simulink model "Unbalanced_Fault_Analysis"  (R2024a)
settings: Solver=VariableStepAuto  StartTime=0.0  StopTime=0.5  RelTol=1e-3
libraries: spsThreePhasePISectionLineLib x2, spsThreePhaseVIMeasurementLib x2, spsThreePhaseParallelRLCLoadLib x1, spsThreePhaseFaultLib x1, spsThreePhaseSourceLib x1, sps_lib x1
settings Model: Creator=Naman V Shetty  LastModifiedBy=Naman V Shetty

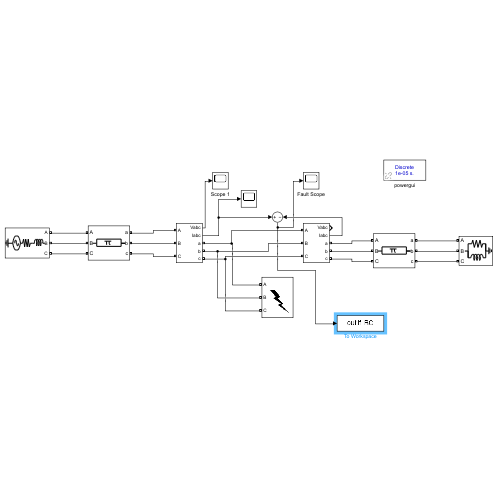
[thumbnail: Simulink's stored preview of the top-level diagram]
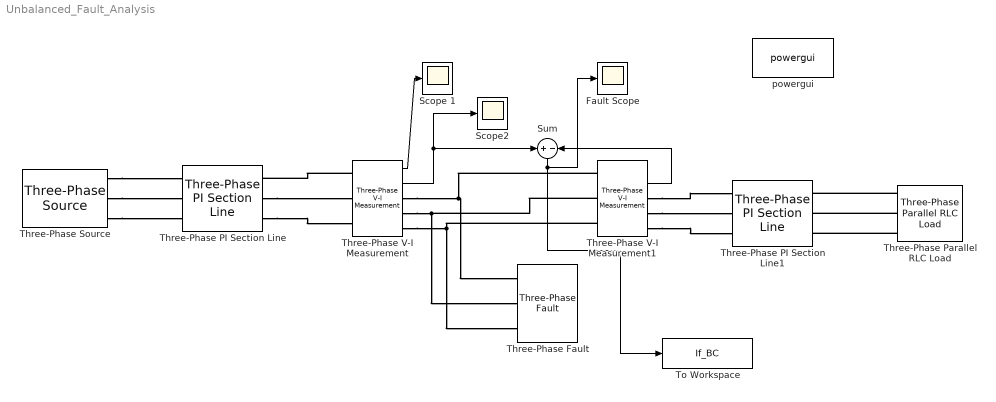
== system Unbalanced_Fault_Analysis ==
  Fault Scope : Scope
  Scope 1 : Scope
      settings: Tag=Voltage
  Scope2 : Scope
  Sum : Sum  Inputs=+-
  Three-Phase PI Section Line : spsThreePhasePISectionLineLib/Three-Phase PI Section Line  LConnTagsString=a|b|c  RConnTagsString=A|B|C  Length=25  Frequency=50  Resistances=[0.2 0.6]  Inductances=[0.001 0.003]  Capacitances=[12e-9 6e-9]
  Three-Phase PI Section Line1 : spsThreePhasePISectionLineLib/Three-Phase PI Section Line  LConnTagsString=a|b|c  RConnTagsString=A|B|C  Length=25  Frequency=50  Resistances=[0.2 0.6]  Inductances=[0.001 0.003]  Capacitances=[12e-9 6e-9]
  Three-Phase Parallel RLC Load : spsThreePhaseParallelRLCLoadLib/Three-Phase Parallel RLC Load  LConnTagsString=A|B|C  Configuration=Y (grounded)  NominalVoltage=11000  Vabc=[1e3 1e3 1e3]  Vabcp=[1e3 1e3 1e3]  NominalFrequency=50  UnbalancedPower=off  ActivePower=1.5e6  InductivePower=0.5e6  CapacitivePower=0  Pabc=[10e3 9e3 11e3]  QLabc=[100 90 110]  QCabc=[100 90 110]  Pabcp=[10e3 9e3 11e3]  QLabcp=[100 90 110]  QCabcp=[100 90 110]  Measurements=None  LoadType=constant Z
  Three-Phase V-I Measurement : spsThreePhaseVIMeasurementLib/Three-Phase V-I Measurement  VoltageMeasurement=phase-to-ground  SetLabelV=off  LabelV=Vabc  Vpu=off  VpuLL=off  CurrentMeasurement=yes  SetLabelI=off  LabelI=Iabc  Ipu=off  Pbase=100e6  Vbase=500e3  OutputType=Complex  PhasorSimulation=off  PSBequivalent=0
  Three-Phase V-I Measurement1 : spsThreePhaseVIMeasurementLib/Three-Phase V-I Measurement  VoltageMeasurement=phase-to-ground  SetLabelV=off  LabelV=Vabc  Vpu=off  VpuLL=off  CurrentMeasurement=yes  SetLabelI=off  LabelI=Iabc  Ipu=off  Pbase=100e6  Vbase=500e3  OutputType=Complex  PhasorSimulation=off  PSBequivalent=0
  Three-Phase Fault : spsThreePhaseFaultLib/Three-Phase Fault  InitialStates=0  FaultA=off  FaultB=on  FaultC=on  GroundFault=off  SwitchTimes=[0.1 0.3]  External=off  SwitchStatus=NaN  FaultResistance=0.01  GroundResistance=0.01  SnubberResistance=1e6  SnubberCapacitance=inf  Measurements=None
  Three-Phase Source : spsThreePhaseSourceLib/Three-Phase Source  InternalConnection=Yg  VoltagePhases=off  Voltage=11000  PhaseAngle=0  Voltage_phases=[25e3 25e3 25e3]/sqrt(3)  PhaseAngles_phases=[0 -120 +120]  Frequency=50  NonIdealSource=on  SpecifyImpedance=off  Resistance=0.1  Inductance=0.001  ShortCircuitLevel=100e6  BaseVoltage=11e3  XRratio=7  BusType=swing  Pref=10e3  Qref=0  Prefabc=[10e3, 10e3, 10e3]  Qrefabc=[0, 0, 0]  Qmin=-inf  Qmax=inf
  To Workspace : ToWorkspace  VariableName=If_BC  SaveFormat=Timeseries  SampleTime=-1
  powergui : sps_lib/powergui  Priority=1  SimulationMode=Discrete  SampleTime=1e-5  frequency=60  Iterations=50  frequencyindice=50  Pbase=100e6  ErrMax=1e-4  UnitsV=kV  UnitsW=MW  buscounter=0  FunctionMessages=off  echomessages=off  EnableUseOfTLC=off  CurrentSourceSwitches=off  DisableSnubberDevices=off  DisableRonSwitches=off  DisableVfSwitches=off  DisplayEquations=off  AutomaticDiscreteSolvers=off  SolverType=Tustin/Backward Euler (TBE)  Interpol=off  ExternalGateDelay=off  methode=off  Ts=100  x0status=blocks  SPID=on  SwTol=0  HookPort=off  NonlinearTolerance=1e-4  nMaxIteration=100  ContinueOnMaxIteration=off  RestoreLinks=warning  ResistiveCurrentMeasurement=off  Frange=[0:2:500]  Ylog=off  Xlog=on  ShowGrid=off  save=off  variable=ZData  structure=0  ZoomFFT=off  StartTime=0.0  cycles=1  DisplayStyle=1  fundamental=60  FreqAxis=off  MaxFrequency=1000  frequencyindicesteady=1  RmsSteady=1  display=off
  wires:
  Three-Phase V-I Measurement/1 -> Scope 1/1
  Three-Phase V-I Measurement/2 -> Scope2/1, Sum/1
  Three-Phase V-I Measurement1/2 -> Sum/2
  Sum/1 -> To Workspace/1, Fault Scope/1
  connections:
  Three-Phase Source/RConn1 -- Three-Phase PI Section Line/LConn1
  Three-Phase Source/RConn2 -- Three-Phase PI Section Line/LConn2
  Three-Phase Source/RConn3 -- Three-Phase PI Section Line/LConn3
  Three-Phase V-I Measurement/LConn1 -- Three-Phase PI Section Line/RConn1
  Three-Phase PI Section Line/RConn2 -- Three-Phase V-I Measurement/LConn2
  Three-Phase PI Section Line/RConn3 -- Three-Phase V-I Measurement/LConn3
  Three-Phase V-I Measurement/RConn1 -- Three-Phase V-I Measurement1/LConn1 -- Three-Phase Fault/LConn1
  Three-Phase V-I Measurement/RConn2 -- Three-Phase V-I Measurement1/LConn2 -- Three-Phase Fault/LConn2
  Three-Phase V-I Measurement/RConn3 -- Three-Phase Fault/LConn3 -- Three-Phase V-I Measurement1/LConn3
  Three-Phase Parallel RLC Load/LConn1 -- Three-Phase PI Section Line1/RConn1
  Three-Phase Parallel RLC Load/LConn2 -- Three-Phase PI Section Line1/RConn2
  Three-Phase Parallel RLC Load/LConn3 -- Three-Phase PI Section Line1/RConn3
  Three-Phase V-I Measurement1/RConn1 -- Three-Phase PI Section Line1/LConn1
  Three-Phase V-I Measurement1/RConn2 -- Three-Phase PI Section Line1/LConn2
  Three-Phase V-I Measurement1/RConn3 -- Three-Phase PI Section Line1/LConn3
